simulink model "Veh_Plant_Model"  (R2026b)
settings: Solver=VariableStepAuto
undefined symbols (not defined in the file): drag, m
settings Model: DataDictionary=Acc_data.sldd  Creator=_The_FooL  LastModifiedBy=_The_FooL
settings SimscapeCC: SimscapeLogType=all  SimscapeNominalValues="[{\"value\":\"1\",\"unit\":\"A\"},{\"value\":\"1\",\"unit\":\"bar\"},{\"value\":\"1\",\"unit\":\"cm^2\"},{\"value\":\"1\",\"unit\":\"cm^3/s\"},{\"value\":\"1\",\"unit\":\"kJ/kg\"},{\"value\":\"1\",\"unit\":\"kW\"},{\"value\":\"1\",\"unit\":\"l\"},{\"value\":\"1\",\"unit\":\"N\"},{\"value\":\"1\",\"unit\":\"N*m\"},{\"value\":\"1\",\"unit\":\"V\"},{\"value\":\"0.001\",\"unit\":\"Wb\"}]"  SimscapeUseEnergyAccounting=off

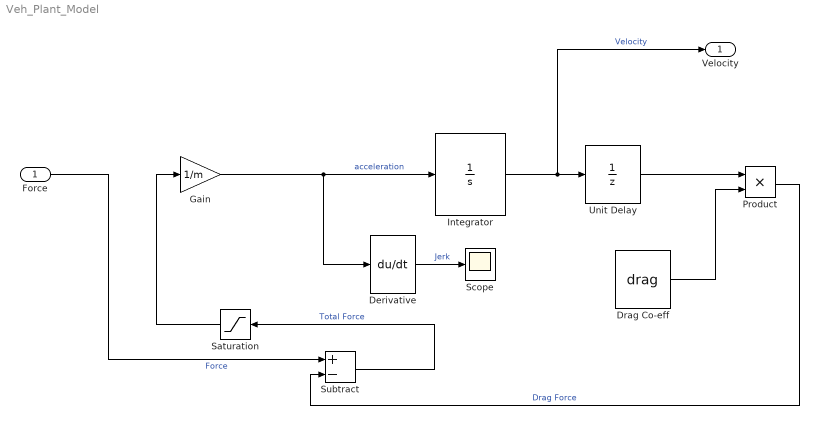
== system Veh_Plant_Model ==
  Force : Inport
  Derivative : Derivative
  Drag Co-eff : Constant  Value=drag
  Gain : Gain  Gain=1/m
  Integrator : Integrator
  Product : Product
  Saturation : Saturate  UpperLimit=9000  LowerLimit=-9000
  Scope : Scope
      settings: ActiveDisplayYMinimum=-0.0815845082608089  ActiveDisplayYMaximum=0.26213012120113743
  Subtract : Sum  Inputs=+-
  Unit Delay : UnitDelay  SampleTime=-1
  Velocity : Outport
  wires:
  Gain/1 -> Derivative/1, Integrator/1  "acceleration"
  Integrator/1 -> Velocity/1, Unit Delay/1  "Velocity"
  Unit Delay/1 -> Product/1
  Drag Co-eff/1 -> Product/2
  Product/1 -> Subtract/2  "Drag Force"
  Derivative/1 -> Scope/1  "Jerk"
  Force/1 -> Subtract/1  "Force"
  Subtract/1 -> Saturation/1  "Total Force"
  Saturation/1 -> Gain/1
